simulink model "InductionHeating_bb_4"  (R2026b)
settings: Solver=FixedStepDiscrete  StopTime=0.008
PostLoadFcn:
  | Ts = 1e-6;Ts_fpga=10e-9;   R=3; Capa=300e-9;L=100e-6;Pejo_factor=1;
InitFcn:
  | Ts = 1e-6;Ts_fpga=10e-9;   R=3; Capa=300e-9;L=100e-6;Pejo_factor=1;
undefined symbols (not defined in the file or in its folder): DiscIntNeverNeededParam, ee_sli_rtmsupport, gcbh, isSetWhenUndefinedState, MATESOCwDio
libraries: fl_lib x67, nesl_utility x40, hdlsllib x32, simulink x15, eeGeneralControl x9, ee_lib x3
(part 4 of 7)

== system InductionHeating_bb_4/MATEwDiode/Diode1 ==
  Pejovic L-C-switch component : Subsystem  AncestorBlock=simetranss/FPGA/Pejovic L-C-switch component  mask(Pejovic Element for FPGA simulation){typ=Switch, Lon=LON, L=1, C=1, traprule=off, otherSW='coming soon', Ts=Ts, pcbp=off, showV=on, showI=on}
      mask prompts: typ "Element type"; Lon "Switch equivalent ON inductance (H)"; L "Inductor inductance (H)"; C "Capacitor capacitance (F)"; traprule "Use Trapezoidal rule (LC only)"; otherSW "Linked Compensated switch name"; Ts "Sample Time (s)"; pcbp "Precharge bypass (inverter only)"; showV "Show voltage port"; showI "Show current port"
      mask help:
      | Pejovic L-C-Switch element  in SimScape
      |
      | Implements either  an inductor, a capacitor or a switch using the Pejovic constant admittance method.
      |
      | For the Switch option, the user only has to select the equivalent ON-state inductance of the model, the corresponding Capacitance is computed internally. In the Pejovic model, Ts/Lon=Coff/Ts (Backward Euler) resulting in a constant admittance for the DAE solver.
      |
      |
      | Input signals;
      |
      | gate: the switch gate value (1 for ON , 0 for OFF) (with Switch option)
      mask init:
      | block=gcb;
      | Xcomp=0;
      | s1=0;s2=0;s3=0;s4=0;r1=0;r2=0;l1=0;l2=0;
      | c1=0;c2=0;c3=0;c4=0;x1=0;x2=0;x3=0;x4=0;
      | 
      | MaskEnables =get_param (block ,'MaskEnables' ); 
      | if isequal(get_param(block,"traprule"),'on')
      |     Trapfactor=2;
      | else
      |     Trapfactor=1;
      | end
      | 
      | if isequal(get_param(block,"showV"),'on')
      |         replace_block (block ,'Followlinks' ,'on' ,'Name' ,'v' ,'BlockType' ,'Terminator' ,'Outport' ,'noprompt' ); 
      | else
      |         replace_block (block ,'Followlinks' ,'on' ,'Name' ,'v' ,'BlockType' ,'Outport' ,'Terminator' ,'noprompt' ); 
      | end
      | if isequal(get_param(block,"showI"),'on')
      |         replace_block (block ,'Followlinks' ,'on' ,'Name' ,'i' ,'BlockType' ,'Terminator' ,'Outport' ,'noprompt' ); 
      | else
      |         replace_block (block ,'Followlinks' ,'on' ,'Name' ,'i' ,'BlockType' ,'Outport' ,'Terminator' ,'noprompt' ); 
      | end
      | 
      | 
      | 
      | 
      | 
      | set_param (block ,'MaskEnables' ,MaskEnables ); 
      | qq='Pejo';
      | 
      | typp=get_param(block,'typ');
      | bp=get_param(block,'pcbp');
      | if isequal(typp,'Switch')
      |     replace_block (block ,'Followlinks' ,'on' ,'Name' ,'gate' ,'BlockType' ,'Constant' ,'Inport' ,'noprompt' ); 
      |     replace_block (block ,'Followlinks' ,'on' ,'Name' ,'init_in' ,'BlockType' ,'Inport' ,'Constant' ,'noprompt'  );
      |     replace_block (block ,'Followlinks' ,'on' ,'Name' ,'init_out' ,'BlockType' ,'Outport' ,'Terminator' ,'noprompt'  );
      |     Rsw=Lon/Ts;
      |     txt='Switch';
      |     [s1,s2,s3,s4,r1,r2,l1,l2,c1,c2,c3,c4] = MATEdrawRLC('Series RLC Branch',0,1,0,'Open circuit');
      |     c2=[0 -20];
      |     c1=[30 120];
      |     qq='Pejo Sw';
      | MaskEnables {2 }='on' ; 
      | MaskEnables {3 }='off' ; 
      | MaskEnables {4 }='off' ; 
      | MaskEnables {5 }='off' ; 
      | MaskEnables {6 }='off' ; 
      | MaskEnables {8 }='off' ;
      | %force Backward Euler
      | set_param(block,'traprule','off');
      |  
      | elseif isequal(typp,'Inductor')
      |     replace_block (block ,'Followlinks' ,'on' ,'Name' ,'gate' ,'BlockType' ,'Inport' ,'Constant' ,'noprompt' ); 
      |     set_param([block '/gate'],'Value','1');
      |     replace_block (block ,'Followlinks' ,'on' ,'Name' ,'init_in' ,'BlockType' ,'Inport' ,'Constant' ,'noprompt'  ); 
      |     replace_block (block ,'Followlinks' ,'on' ,'Name' ,'init_out' ,'BlockType' ,'Outport' ,'Terminator' ,'noprompt'  );
      |     Rsw=L/Ts*Trapfactor;
      |     txt='L';
      |     qq='Pejo L';
      | MaskEnables {2 }='off' ; 
      | MaskEnables {3 }='on' ; 
      | MaskEnables {4 }='off' ; 
      | MaskEnables {5 }='on' ; 
      | MaskEnables {6 }='off' ; 
      | MaskEnables {8 }='off' ;
      |     x1=0;x2=0;x3=0;x4=0;
      |     [s1,s2,s3,s4,r1,r2,l1,l2,c1,c2,c3,c4] = MATEdrawRLC('Series RLC Branch',0,1,0,'L');
      |     
      | elseif isequal(typp,'Capacitor')
      |     replace_block (block ,'Followlinks' ,'on' ,'Name' ,'gate' ,'BlockType' ,'Inport' ,'Constant' ,'noprompt' ); 
      |     set_param([block '/gate'],'Value','0');
      |     replace_block (block ,'Followlinks' ,'on' ,'Name' ,'init_in' ,'BlockType' ,'Inport' ,'Constant' ,'noprompt'  );
      |     replace_block (block ,'Followlinks' ,'on' ,'Name' ,'init_out' ,'BlockType' ,'Outport' ,'Terminator' ,'noprompt'  );
      |     Rsw=Ts/C/Trapfactor;
      |     txt='C';
      |     qq='Pejo C';
      | MaskEnables {2 }='off' ; 
      | MaskEnables {3 }='off' ; 
      | MaskEnables {4 }='on' ; 
      | MaskEnables {5 }='on' ; 
      | MaskEnables {6 }='off' ; 
      | MaskEnables {8 }='off' ;
      |         x1=0;x2=0;x3=0;x4=0;
      |     [s1,s2,s3,s4,r1,r2,l1,l2,c1,c2,c3,c4] = MATEdrawRLC('Series RLC Branch',0,0,1,'C');
      | elseif isequal(typp,'2-level inverter switch')
      |     replace_block (block ,'Followlinks' ,'on' ,'Name' ,'gate' ,'BlockType' ,'Constant' ,'Inport' ,'noprompt' ); 
      |     replace_block (block ,'Followlinks' ,'on' ,'Name' ,'init_in' ,'BlockType' ,'Constant' ,'Inport','noprompt'  );
      |     replace_block (block ,'Followlinks' ,'on' ,'Name' ,'init_out' ,'BlockType' ,'Terminator' ,'Outport' ,'noprompt'  );
      |     Rsw=Lon/Ts;
      |     txt='Inverter half';
      |     Xcomp=1;
      |     qq='Pejo Inverter Half';
      |     %force Backward Euler
      | set_param(block,'traprule','off');
      | MaskEnables {2 }='on' ; 
      | MaskEnables {3 }='off' ; 
      | MaskEnables {4 }='off' ; 
      | MaskEnables {5 }='off' ; 
      | MaskEnables {6 }='off' ; 
      | MaskEnables {8 }='on' ;
      |         [s1,s2,s3,s4,r1,r2,l1,l2,c1,c2,c3,c4] = MATEdrawRLC('Series RLC Branch',0,1,0,'Open circuit');
      |     c2=[0 -20];
      |     c1=[30 120];
      | 
      | else
      | end
      | 
      | if isequal(typp,'2-level inverter switch')  && isequal(bp,'on')
      |         replace_block (block ,'Followlinks' ,'on' ,'Name' ,'Bypass' ,'BlockType' ,'Ground' ,'Inport' ,'noprompt' ); 
      | else
      |         replace_block (block ,'Followlinks' ,'on' ,'Name' ,'Bypass' ,'BlockType' ,'Inport' ,'Ground' ,'noprompt' ); 
      | end
      | 
      | MaskEnables {7 }='on' ; 
      | set_param (block ,'MaskEnables' ,MaskEnables ); 
      | 
      | 
      | if Ts>2e-6
      |     %warndlg(['Sample Time of ' num2str(Ts) ' s. may be somehow large for the Pejovic switch to be accurate. Sample time below 2 us are recommended.'])
      | end
      mask TypeOptions typ: Switch | Inductor | Capacitor | 2-level inverter switch
      mask Display:
      | plot(s1,s2,s3,s4,r1,r2,l1,l2,c1,c2,c3,c4,x1,x2,x3,x4);
      | color('blue')
      | port_label('LConn',1,'+')
      | disp([qq  10 10])
  Relational Operator : RelationalOperator  Operator=>  OutDataTypeStr=boolean  RndMeth=Simplest  InputSameDT=off
  Relational Operator1 : RelationalOperator  Operator=>  OutDataTypeStr=boolean  RndMeth=Simplest  InputSameDT=off
  Resistor1 : fl_lib/Electrical/Electrical Elements/Resistor  R=RON Ohm  i_specify=off  i_priority=None  i=0 A  i_nominal_specify=off  i_nominal_value=1  i_nominal_unit=A  v_specify=off  v_priority=None  v=0 V  v_nominal_specify=off  v_nominal_value=1  v_nominal_unit=V
  Set-Reset Flip-Flop : eeGeneralControl/Set-Reset Flip-Flop  LabelModeActiveChoice=Discrete  UndefState=Set  Q0=0  Ts=Ts
  Terminator : Terminator
  Unit Delay : UnitDelay  SampleTime=Ts
  Vf : Constant  Value=0  SampleTime=Ts
  Vf2 : Constant  Value=VF  SampleTime=Ts
  currrent OFF : Constant  Value=0  SampleTime=Ts
  +V : PMIOPort  Side=Left
  -V : PMIOPort  Port=2  Side=Right
  wires:
  Vf2/1 -> Pejovic L-C-switch component/2(Vf)
  Relational Operator/1 -> Set-Reset Flip-Flop/1
  Set-Reset Flip-Flop/1 -> Unit Delay/1
  Unit Delay/1 -> Pejovic L-C-switch component/1(gate)
  Relational Operator1/1 -> Set-Reset Flip-Flop/2
  currrent OFF/1 -> Relational Operator1/2
  Set-Reset Flip-Flop/2 -> Terminator/1
  Vf/1 -> Relational Operator/2
  Pejovic L-C-switch component/2(i) -> Relational Operator1/1
  Pejovic L-C-switch component/1(v) -> Relational Operator/1
  connections:
  Resistor1/RConn1 -- +V/RConn1
  Pejovic L-C-switch component/RConn1 -- -V/RConn1
  Resistor1/LConn1 -- Pejovic L-C-switch component/LConn1

== system InductionHeating_bb_4/MATEwDiode/Diode2 ==
  Pejovic L-C-switch component : Subsystem  AncestorBlock=simetranss/FPGA/Pejovic L-C-switch component  mask(Pejovic Element for FPGA simulation){typ=Switch, Lon=LON, L=1, C=1, traprule=off, otherSW='coming soon', Ts=Ts, pcbp=off, showV=on, showI=on}
      mask prompts: typ "Element type"; Lon "Switch equivalent ON inductance (H)"; L "Inductor inductance (H)"; C "Capacitor capacitance (F)"; traprule "Use Trapezoidal rule (LC only)"; otherSW "Linked Compensated switch name"; Ts "Sample Time (s)"; pcbp "Precharge bypass (inverter only)"; showV "Show voltage port"; showI "Show current port"
      mask help:
      | Pejovic L-C-Switch element  in SimScape
      |
      | Implements either  an inductor, a capacitor or a switch using the Pejovic constant admittance method.
      |
      | For the Switch option, the user only has to select the equivalent ON-state inductance of the model, the corresponding Capacitance is computed internally. In the Pejovic model, Ts/Lon=Coff/Ts (Backward Euler) resulting in a constant admittance for the DAE solver.
      |
      |
      | Input signals;
      |
      | gate: the switch gate value (1 for ON , 0 for OFF) (with Switch option)
      mask init: same as InductionHeating_bb_4/MATEwDiode/Diode1/Pejovic L-C-switch component
      mask TypeOptions typ: Switch | Inductor | Capacitor | 2-level inverter switch
      mask Display:
      | plot(s1,s2,s3,s4,r1,r2,l1,l2,c1,c2,c3,c4,x1,x2,x3,x4);
      | color('blue')
      | port_label('LConn',1,'+')
      | disp([qq  10 10])
  Relational Operator : RelationalOperator  Operator=>  OutDataTypeStr=boolean  RndMeth=Simplest  InputSameDT=off
  Relational Operator1 : RelationalOperator  Operator=>  OutDataTypeStr=boolean  RndMeth=Simplest  InputSameDT=off
  Resistor1 : fl_lib/Electrical/Electrical Elements/Resistor  R=RON Ohm  i_specify=off  i_priority=None  i=0 A  i_nominal_specify=off  i_nominal_value=1  i_nominal_unit=A  v_specify=off  v_priority=None  v=0 V  v_nominal_specify=off  v_nominal_value=1  v_nominal_unit=V
  Set-Reset Flip-Flop : eeGeneralControl/Set-Reset Flip-Flop  LabelModeActiveChoice=Discrete  UndefState=Set  Q0=0  Ts=Ts
  Terminator : Terminator
  Unit Delay : UnitDelay  SampleTime=Ts
  Vf : Constant  Value=0  SampleTime=Ts
  Vf2 : Constant  Value=VF  SampleTime=Ts
  currrent OFF : Constant  Value=0  SampleTime=Ts
  +V : PMIOPort  Side=Left
  -V : PMIOPort  Port=2  Side=Right
  wires:
  Pejovic L-C-switch component/1(v) -> Relational Operator/1
  Pejovic L-C-switch component/2(i) -> Relational Operator1/1
  Vf/1 -> Relational Operator/2
  Set-Reset Flip-Flop/2 -> Terminator/1
  currrent OFF/1 -> Relational Operator1/2
  Relational Operator1/1 -> Set-Reset Flip-Flop/2
  Unit Delay/1 -> Pejovic L-C-switch component/1(gate)
  Set-Reset Flip-Flop/1 -> Unit Delay/1
  Relational Operator/1 -> Set-Reset Flip-Flop/1
  Vf2/1 -> Pejovic L-C-switch component/2(Vf)
  connections:
  Resistor1/LConn1 -- Pejovic L-C-switch component/LConn1
  Pejovic L-C-switch component/RConn1 -- -V/RConn1
  Resistor1/RConn1 -- +V/RConn1

== system InductionHeating_bb_4/MATEwDiode/Diode3 ==
  Pejovic L-C-switch component : Subsystem  AncestorBlock=simetranss/FPGA/Pejovic L-C-switch component  mask(Pejovic Element for FPGA simulation){typ=Switch, Lon=LON, L=1, C=1, traprule=off, otherSW='coming soon', Ts=Ts, pcbp=off, showV=on, showI=on}
      mask prompts: typ "Element type"; Lon "Switch equivalent ON inductance (H)"; L "Inductor inductance (H)"; C "Capacitor capacitance (F)"; traprule "Use Trapezoidal rule (LC only)"; otherSW "Linked Compensated switch name"; Ts "Sample Time (s)"; pcbp "Precharge bypass (inverter only)"; showV "Show voltage port"; showI "Show current port"
      mask help:
      | Pejovic L-C-Switch element  in SimScape
      |
      | Implements either  an inductor, a capacitor or a switch using the Pejovic constant admittance method.
      |
      | For the Switch option, the user only has to select the equivalent ON-state inductance of the model, the corresponding Capacitance is computed internally. In the Pejovic model, Ts/Lon=Coff/Ts (Backward Euler) resulting in a constant admittance for the DAE solver.
      |
      |
      | Input signals;
      |
      | gate: the switch gate value (1 for ON , 0 for OFF) (with Switch option)
      mask init: same as InductionHeating_bb_4/MATEwDiode/Diode1/Pejovic L-C-switch component
      mask TypeOptions typ: Switch | Inductor | Capacitor | 2-level inverter switch
      mask Display:
      | plot(s1,s2,s3,s4,r1,r2,l1,l2,c1,c2,c3,c4,x1,x2,x3,x4);
      | color('blue')
      | port_label('LConn',1,'+')
      | disp([qq  10 10])
  Relational Operator : RelationalOperator  Operator=>  OutDataTypeStr=boolean  RndMeth=Simplest  InputSameDT=off
  Relational Operator1 : RelationalOperator  Operator=>  OutDataTypeStr=boolean  RndMeth=Simplest  InputSameDT=off
  Resistor1 : fl_lib/Electrical/Electrical Elements/Resistor  R=RON Ohm  i_specify=off  i_priority=None  i=0 A  i_nominal_specify=off  i_nominal_value=1  i_nominal_unit=A  v_specify=off  v_priority=None  v=0 V  v_nominal_specify=off  v_nominal_value=1  v_nominal_unit=V
  Set-Reset Flip-Flop : eeGeneralControl/Set-Reset Flip-Flop  LabelModeActiveChoice=Discrete  UndefState=Set  Q0=0  Ts=Ts
  Terminator : Terminator
  Unit Delay : UnitDelay  SampleTime=Ts
  Vf : Constant  Value=0  SampleTime=Ts
  Vf2 : Constant  Value=VF  SampleTime=Ts
  currrent OFF : Constant  Value=0  SampleTime=Ts
  +V : PMIOPort  Side=Left
  -V : PMIOPort  Port=2  Side=Right
  wires:
  Pejovic L-C-switch component/1(v) -> Relational Operator/1
  Pejovic L-C-switch component/2(i) -> Relational Operator1/1
  Vf/1 -> Relational Operator/2
  Set-Reset Flip-Flop/2 -> Terminator/1
  currrent OFF/1 -> Relational Operator1/2
  Relational Operator1/1 -> Set-Reset Flip-Flop/2
  Unit Delay/1 -> Pejovic L-C-switch component/1(gate)
  Set-Reset Flip-Flop/1 -> Unit Delay/1
  Relational Operator/1 -> Set-Reset Flip-Flop/1
  Vf2/1 -> Pejovic L-C-switch component/2(Vf)
  connections:
  Resistor1/LConn1 -- Pejovic L-C-switch component/LConn1
  Pejovic L-C-switch component/RConn1 -- -V/RConn1
  Resistor1/RConn1 -- +V/RConn1

== system InductionHeating_bb_4/MATEwDiode/Diode4 ==
  Pejovic L-C-switch component : Subsystem  AncestorBlock=simetranss/FPGA/Pejovic L-C-switch component  mask(Pejovic Element for FPGA simulation){typ=Switch, Lon=LON, L=1, C=1, traprule=off, otherSW='coming soon', Ts=Ts, pcbp=off, showV=on, showI=on}
      mask prompts: typ "Element type"; Lon "Switch equivalent ON inductance (H)"; L "Inductor inductance (H)"; C "Capacitor capacitance (F)"; traprule "Use Trapezoidal rule (LC only)"; otherSW "Linked Compensated switch name"; Ts "Sample Time (s)"; pcbp "Precharge bypass (inverter only)"; showV "Show voltage port"; showI "Show current port"
      mask help:
      | Pejovic L-C-Switch element  in SimScape
      |
      | Implements either  an inductor, a capacitor or a switch using the Pejovic constant admittance method.
      |
      | For the Switch option, the user only has to select the equivalent ON-state inductance of the model, the corresponding Capacitance is computed internally. In the Pejovic model, Ts/Lon=Coff/Ts (Backward Euler) resulting in a constant admittance for the DAE solver.
      |
      |
      | Input signals;
      |
      | gate: the switch gate value (1 for ON , 0 for OFF) (with Switch option)
      mask init: same as InductionHeating_bb_4/MATEwDiode/Diode1/Pejovic L-C-switch component
      mask TypeOptions typ: Switch | Inductor | Capacitor | 2-level inverter switch
      mask Display:
      | plot(s1,s2,s3,s4,r1,r2,l1,l2,c1,c2,c3,c4,x1,x2,x3,x4);
      | color('blue')
      | port_label('LConn',1,'+')
      | disp([qq  10 10])
  Relational Operator : RelationalOperator  Operator=>  OutDataTypeStr=boolean  RndMeth=Simplest  InputSameDT=off
  Relational Operator1 : RelationalOperator  Operator=>  OutDataTypeStr=boolean  RndMeth=Simplest  InputSameDT=off
  Resistor1 : fl_lib/Electrical/Electrical Elements/Resistor  R=RON Ohm  i_specify=off  i_priority=None  i=0 A  i_nominal_specify=off  i_nominal_value=1  i_nominal_unit=A  v_specify=off  v_priority=None  v=0 V  v_nominal_specify=off  v_nominal_value=1  v_nominal_unit=V
  Set-Reset Flip-Flop : eeGeneralControl/Set-Reset Flip-Flop  LabelModeActiveChoice=Discrete  UndefState=Set  Q0=0  Ts=Ts
  Terminator : Terminator
  Unit Delay : UnitDelay  SampleTime=Ts
  Vf : Constant  Value=0  SampleTime=Ts
  Vf2 : Constant  Value=VF  SampleTime=Ts
  currrent OFF : Constant  Value=0  SampleTime=Ts
  +V : PMIOPort  Side=Left
  -V : PMIOPort  Port=2  Side=Right
  wires:
  Vf2/1 -> Pejovic L-C-switch component/2(Vf)
  Relational Operator/1 -> Set-Reset Flip-Flop/1
  Set-Reset Flip-Flop/1 -> Unit Delay/1
  Unit Delay/1 -> Pejovic L-C-switch component/1(gate)
  Relational Operator1/1 -> Set-Reset Flip-Flop/2
  currrent OFF/1 -> Relational Operator1/2
  Set-Reset Flip-Flop/2 -> Terminator/1
  Vf/1 -> Relational Operator/2
  Pejovic L-C-switch component/2(i) -> Relational Operator1/1
  Pejovic L-C-switch component/1(v) -> Relational Operator/1
  connections:
  Resistor1/RConn1 -- +V/RConn1
  Pejovic L-C-switch component/RConn1 -- -V/RConn1
  Resistor1/LConn1 -- Pejovic L-C-switch component/LConn1

== system InductionHeating_bb_4/MATEwDiode/MATE 2-level inverter ==
  g : Inport
  CCS_Idc : fl_lib/Electrical/Electrical Sources/Controlled Current Source
  CVS : fl_lib/Electrical/Electrical Sources/Controlled Voltage Source
  Constant : Constant  Value=[Gpp Ts/Gip min_charge Vf]  SampleTime=Ts
  Isensor : fl_lib/Electrical/Electrical Sensors/Current Sensor
  PS-Simulink Converter : nesl_utility/PS-Simulink Converter  PhysicalDomain=network_engine_domain  SubClassName=ps_output  LeftPortType=input  RightPortType=output  PseudoPeriodic=off  Frequencies=[]  VectorFormat=inherit  Unit=inherit  AffineConversion=off
  PS-Simulink Converter1 : nesl_utility/PS-Simulink Converter  PhysicalDomain=network_engine_domain  SubClassName=ps_output  LeftPortType=input  RightPortType=output  PseudoPeriodic=off  Frequencies=[]  VectorFormat=inherit  Unit=inherit  AffineConversion=off
  R : fl_lib/Electrical/Electrical Elements/Resistor  R=Ron Ohm  i_specify=off  i_priority=None  i=0 A  i_nominal_specify=off  i_nominal_value=1  i_nominal_unit=A  v_specify=off  v_priority=None  v=0 V  v_nominal_specify=off  v_nominal_value=1  v_nominal_unit=V
  SW : Subsystem
  Selector : Selector  InputPortWidth=2  IndexOptions=Index vector (dialog)  Indices=[1 ]  OutputSizes=1  RuntimeRangeChecks=off
  Selector1 : Selector  InputPortWidth=2  IndexOptions=Index vector (dialog)  Indices=[2 ]  OutputSizes=1  RuntimeRangeChecks=off
  Simulink-PS Converter : nesl_utility/Simulink-PS Converter  PhysicalDomain=network_engine_domain  SubClassName=ps_input  LeftPortType=input  RightPortType=output  PseudoPeriodic=off  Frequencies=[]  NoiseDistribution=none  NoiseParameters=[]  Unit=1  AffineConversion=off  FilteringAndDerivatives=provide  SimscapeFilterOrder=1  InputFilterTimeConstant=0.001  UdotUserProvided=0
  Simulink-PS Converter1 : nesl_utility/Simulink-PS Converter  PhysicalDomain=network_engine_domain  SubClassName=ps_input  LeftPortType=input  RightPortType=output  PseudoPeriodic=off  Frequencies=[]  NoiseDistribution=none  NoiseParameters=[]  Unit=1  AffineConversion=off  FilteringAndDerivatives=provide  SimscapeFilterOrder=1  InputFilterTimeConstant=0.001  UdotUserProvided=0
  Unit Delay2 : UnitDelay  SampleTime=Ts
  Unit Delay3 : UnitDelay  SampleTime=Ts
  Vsensor : fl_lib/Electrical/Electrical Sensors/Voltage Sensor
  V+ : PMIOPort  Side=Left
  V- : PMIOPort  Port=2  Side=Left
  A : PMIOPort  Port=3  Side=Right
  wires:
  SW/2(Vac) -> Simulink-PS Converter1/1
  Constant/1 -> SW/5(params)
  Unit Delay3/1 -> SW/3(Vdc)
  Unit Delay2/1 -> SW/4(Iac)
  SW/1(Idc) -> Simulink-PS Converter/1
  g/1 -> Selector/1, Selector1/1
  PS-Simulink Converter1/1 -> Unit Delay3/1
  PS-Simulink Converter/1 -> Unit Delay2/1
  Selector/1 -> SW/1(gu)
  Selector1/1 -> SW/2(gl)
  connections:
  Isensor/RConn2 -- CVS/LConn1
  R/LConn1 -- Isensor/LConn1
  Simulink-PS Converter/RConn1 -- CCS_Idc/RConn1
  PS-Simulink Converter/LConn1 -- Isensor/RConn1
  Simulink-PS Converter1/RConn1 -- CVS/RConn1
  CCS_Idc/LConn1 -- Vsensor/RConn2 -- V-/RConn1 -- CVS/RConn2
  CCS_Idc/RConn2 -- Vsensor/LConn1 -- V+/RConn1
  PS-Simulink Converter1/LConn1 -- Vsensor/RConn1
  A/RConn1 -- R/RConn1

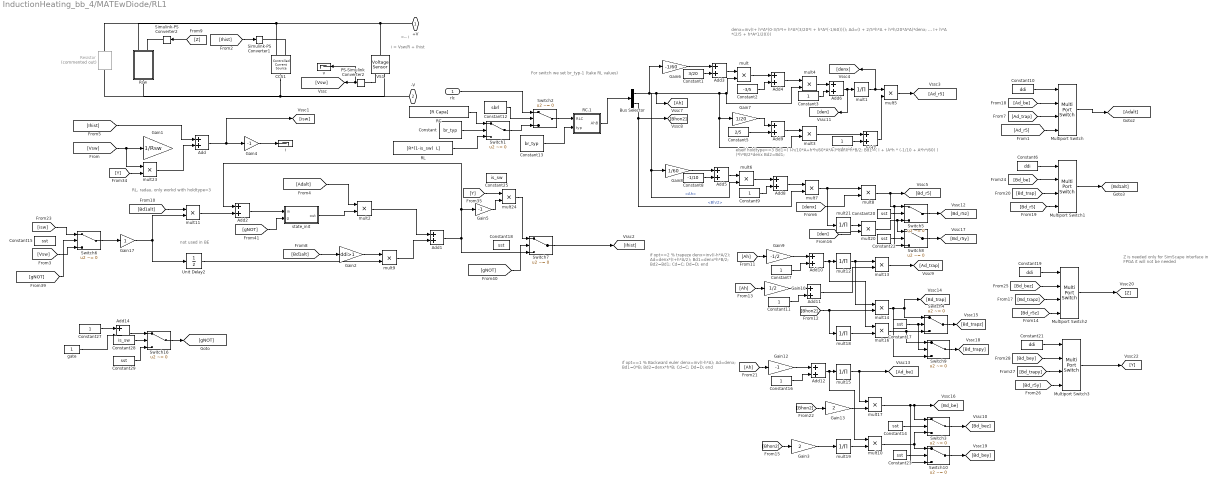
== system InductionHeating_bb_4/MATEwDiode/RL1 ==
  note: For switch we set br_typ-1 (take RL values)
  note: if opt==1 % Backward euler
      | denx=inv(I-h*A);
      | Ad=denx;
      | Bd1=0*B;
      | Bd2=denx*h*B;
      | Cd=C;
      | Dd=D;
      | end
  note: if opt==2 % trapeze
      | denx=inv(I-h*A/2);
      | Ad=denx*(I+h*A/2);
      | Bd1=denx*h*B/2;
      | Bd2=Bd1;
      | Cd=C;
      | Dd=D;
      | end
  note: RL, radau, only workd with holdtype=3
  note: elseif holdtype==3
      | Bd1=( I-h/10*A+h*h/60*A*A )*denx*h*B/2;
      | Bd1=( I + (A*h * (-1/10 + A*h*/60) ) )*h*B/2*denx
      | Bd2=Bd1;
  note: denx=inv(I+ h*A*(0-3/5*I+ h*A*(3/20*I + h*A*(-1/60))));
      | Ad=(I + 2/5*h*A + h*h/20*A*A)*denx;
      | ... I+ h*A *(2/5 + h*A*1/20)))
  note: <-- i
  note: i = Vsw/R + Ihist
  note: Z is needed only for SimScape interface
      | in FPGA it will not be needed
  note: not used in BE
  rlc : Inport
  Add : Sum
  Add{1..12} (12 alike) : Sum  Inputs=2
  Add14 : Sum  Inputs=+-
  Bus Selector : BusSelector  OutputSignals=Ah,Bh/2
  CCS1 : fl_lib/Electrical/Electrical Sources/Controlled Current Source
  Constant : Constant  Value=br_typ
  Constant1 : Constant  Value=3/20  SampleTime=Ts
  Constant{6,10,19,21} (4 alike) : Constant  Value=ddi  SampleTime=Ts
  Constant{3..4,7,9,11,16,27} (7 alike) : Constant  SampleTime=Ts
  Constant12 : Constant  Value=sbrl
  Constant13 : Constant  Value=br_typ
  Constant{14..15,17..18,20,22..23,29} (8 alike) : Constant  Value=sst  SampleTime=Ts
  Constant2 : Constant  Value=-3/5  SampleTime=Ts
  Constant25 : Constant  Value=is_sw  SampleTime=Ts
  Constant28 : Constant  Value=is_sw  SampleTime=Ts
  Constant5 : Constant  Value=2/5  SampleTime=Ts
  Constant8 : Constant  Value=-1/10  SampleTime=Ts
  Gain1 : Gain  Gain=1/Rsw
  Gain10 : Gain  Gain=1/2
  Gain12 : Gain  Gain=-1
  Gain13 : Gain  Gain=2
  Gain17 : Gain
  Gain2 : Gain  Gain=ddi>1
  Gain3 : Gain  Gain=2
  Gain4 : Gain  Gain=-1
  Gain5 : Gain  Gain=-1
  Gain6 : Gain  Gain=-1/60
  Gain7 : Gain  Gain=1/20
  Gain8 : Gain  Gain=1/60
  Gain9 : Gain  Gain=-1/2
  Multiport Switch{,1..3} (4 alike) : MultiPortSwitch  SaturateOnIntegerOverflow=off  InputSameDT=off
  PS-Simulink Converter2 : nesl_utility/PS-Simulink Converter  PhysicalDomain=network_engine_domain  SubClassName=ps_output  LeftPortType=input  RightPortType=output  PseudoPeriodic=off  Frequencies=[]  VectorFormat=inherit  Unit=inherit  AffineConversion=off
  RC : Constant  Value=[R Capa]  SampleTime=Ts
  RC.1 : Subsystem
  RL : Constant  Value="[R*(1-is_sw)  L]"  SampleTime=Ts
  Resistor : fl_lib/Electrical/Electrical Elements/Resistor  Commented=on  R=Rsw Ohm  i_specify=off  i_priority=None  i=0 A  i_nominal_specify=off  i_nominal_value=1  i_nominal_unit=A  v_specify=off  v_priority=None  v=0 V  v_nominal_specify=off  v_nominal_value=1  v_nominal_unit=V
  Rsw : Subsystem  mask(Simscape MATE variable resistance default value mask){defaultR=Rsw}
      mask prompts: defaultR "Default Resistance"
  Simulink-PS Converter1 : nesl_utility/Simulink-PS Converter  PhysicalDomain=network_engine_domain  SubClassName=ps_input  LeftPortType=input  RightPortType=output  PseudoPeriodic=off  Frequencies=[]  NoiseDistribution=none  NoiseParameters=[]  Unit=1  AffineConversion=off  FilteringAndDerivatives=provide  SimscapeFilterOrder=1  InputFilterTimeConstant=0.001  UdotUserProvided=0
  Simulink-PS Converter2 : nesl_utility/Simulink-PS Converter  PhysicalDomain=network_engine_domain  SubClassName=ps_input  LeftPortType=input  RightPortType=output  PseudoPeriodic=off  Frequencies=[]  NoiseDistribution=none  NoiseParameters=[]  Unit=1  AffineConversion=off  FilteringAndDerivatives=provide  SimscapeFilterOrder=1  InputFilterTimeConstant=0.001  UdotUserProvided=0
  Switch{1..10} (10 alike) : Switch  Criteria=u2 ~= 0  SaturateOnIntegerOverflow=off  InputSameDT=off
  Switch16 : Switch  Criteria=u2 ~= 0  Threshold=0.5  SaturateOnIntegerOverflow=off  InputSameDT=off
  Unit Delay2 : UnitDelay  SampleTime=-1
  VS1 : fl_lib/Electrical/Electrical Sensors/Voltage Sensor
  gate : Constant
  i : Terminator
  mult{,2..11,13..14,16..17,20,23..24} (18 alike) : Product
  mult{1,12,15,18..19,21} (6 alike) : Product  Inputs=/
  state_init : Subsystem
  v : Terminator
  +V : PMIOPort  Side=Left
  -V : PMIOPort  Port=2  Side=Right
  wires:
  Constant29/1 -> Switch16/3
  Constant28/1 -> Switch16/2
  Switch16/1 -> [gNOT]
  Add14/1 -> Switch16/1
  [gNOT] -> state_init/2(g)
  state_init/1(out) -> mult2/2
  [gNOT] -> Switch7/2
  [gNOT] -> Switch6/2
  Constant27/1 -> Add14/1
  Gain17/1 -> Unit Delay2/1, mult11/2
  Gain5/1 -> mult24/2
  [Y] -> mult24/1
  mult24/1 -> Switch7/1
  mult23/1 -> Add/2
  [Y] -> mult23/2
  Multiport Switch3/1 -> [Y]
  Constant23/1 -> Switch10/2
  Switch10/1 -> [Bd_bey]
  mult14/1 -> Switch4/1, [Bd_trap], Switch9/3
  mult16/1 -> Switch4/3, Switch9/1
  Constant17/1 -> Switch4/2, Switch9/2
  Switch9/1 -> [Bd_trapy]
  Constant22/1 -> Switch8/2
  Switch8/1 -> [Bd_r5y]
  [Bd_r5y] -> Multiport Switch3/4
  [Bd_trapy] -> Multiport Switch3/3
  [Bd_bey] -> Multiport Switch3/2
  Constant21/1 -> Multiport Switch3/1
  Switch4/1 -> [Bd_trapz]
  mult8/1 -> Switch5/1, Switch8/3, [Bd_r5]
  Constant19/1 -> Multiport Switch2/1
  Multiport Switch2/1 -> [Z]
  [Bd_bez] -> Multiport Switch2/2
  [Bd_trapz] -> Multiport Switch2/3
  [Bd_r5z] -> Multiport Switch2/4
  mult2/1 -> Add1/1
  [isw] -> Switch6/1
  [Vsw] -> Switch6/3
  Switch6/1 -> Gain17/1
  Add/1 -> Gain4/1, [isw]
  [Ihist] -> Simulink-PS Converter1/1
  [Vsw] -> Gain1/1, mult23/1
  PS-Simulink Converter2/1 -> v/1, [Vsw]
  [Ihist] -> Add/1
  Gain4/1 -> i/1
  Add2/1 -> state_init/1(in)
  Add1/1 -> Add2/1, Gain5/1, Switch7/3
  Unit Delay2/1 -> mult9/2
  Gain6/1 -> Add3/1
  Constant1/1 -> Add3/2
  mult/1 -> Add4/1
  Add3/1 -> mult/1
  Constant2/1 -> Add4/2
  Add4/1 -> mult4/1
  mult4/1 -> Add6/1
  Constant3/1 -> Add6/2
  Add6/1 -> [den], mult1/1
  Constant4/1 -> Add7/2
  Constant5/1 -> Add9/2
  Add9/1 -> mult3/1
  Gain7/1 -> Add9/1
  mult3/1 -> Add7/1
  Add7/1 -> mult5/2
  [Adalt] -> mult2/1
  mult1/1 -> [denx], mult5/1
  mult5/1 -> [Ad_r5]
  Constant9/1 -> Add8/2
  Add5/1 -> mult6/1
  mult6/1 -> Add8/1
  Constant8/1 -> Add5/2
  Gain8/1 -> Add5/1
  Add8/1 -> mult7/1
  mult7/1 -> mult21/1, mult8/1
  [denx] -> mult8/2
  Bus Selector/1 -> Gain6/1, [Ah], mult3/2, Gain7/1, mult4/2, mult/2, Gain8/1, mult6/2  "<Ah>"
  Bus Selector/2 -> mult7/2, [Bhon2]  "<Bh/2>"
  [Z] -> Simulink-PS Converter2/1
  [Ah] -> Gain9/1
  Gain9/1 -> Add10/1
  Constant7/1 -> Add10/2
  Add10/1 -> mult16/1, mult12/1
  Add11/1 -> mult13/2
  Constant11/1 -> Add11/2
  Gain10/1 -> Add11/1
  [Ah] -> Gain10/1
  mult12/1 -> mult14/1, mult13/1
  [Bhon2] -> mult18/1, mult14/2
  mult13/1 -> [Ad_trap]
  mult9/1 -> Add1/2
  [Bd1alt] -> Gain2/1
  [Bd1alt] -> mult11/1
  mult11/1 -> Add2/2
  mult15/1 -> [Ad_be], mult17/1
  [Bhon2] -> Gain13/1
  Add12/1 -> mult10/1, mult15/1
  Constant16/1 -> Add12/2
  Gain12/1 -> Add12/1
  [Ah] -> Gain12/1
  Gain13/1 -> mult17/2
  [Ad_r5] -> Multiport Switch/4
  [Ad_trap] -> Multiport Switch/3
  [Ad_be] -> Multiport Switch/2
  Multiport Switch/1 -> [Adalt]
  [Bd_r5] -> Multiport Switch1/4
  [Bd_trap] -> Multiport Switch1/3
  [Bd_be] -> Multiport Switch1/2
  Multiport Switch1/1 -> [Bd1alt]
  Constant6/1 -> Multiport Switch1/1
  Constant10/1 -> Multiport Switch/1
  Gain2/1 -> mult9/1
  RC/1 -> Switch1/1
  RL/1 -> Switch1/3
  Constant/1 -> Switch1/2
  Switch1/1 -> Switch2/3
  Switch2/1 -> RC.1/1(RLC)
  rlc/1 -> Switch2/1
  Constant12/1 -> Switch2/2
  RC.1/1(AhB) -> Bus Selector/1
  Constant13/1 -> RC.1/2(typ)
  mult18/1 -> mult16/2
  Gain3/1 -> mult19/1
  [Bhon2] -> Gain3/1
  mult19/1 -> mult10/2
  mult10/1 -> Switch3/3, Switch10/1
  mult17/1 -> Switch3/1, [Bd_be], Switch10/3
  Constant14/1 -> Switch3/2
  Switch3/1 -> [Bd_bez]
  [den] -> mult20/2
  mult21/1 -> mult20/1
  Switch5/1 -> [Bd_r5z]
  Constant20/1 -> Switch5/2
  mult20/1 -> Switch5/3, Switch8/1
  gate/1 -> Add14/2
  Switch7/1 -> [Ihist]
  connections:
  CCS1/RConn2 -- +V/RConn1 -- VS1/LConn1 -- Resistor/LConn1 -- Rsw/LConn1
  CCS1/RConn1 -- Simulink-PS Converter1/RConn1
  PS-Simulink Converter2/LConn1 -- VS1/RConn1
  CCS1/LConn1 -- -V/RConn1 -- VS1/RConn2 -- Resistor/RConn1 -- Rsw/RConn1
  Simulink-PS Converter2/RConn1 -- Rsw/LConn2

== system InductionHeating_bb_4/MATEwDiode/Subsystem3 ==
  ILoad : fl_lib/Electrical/Electrical Sensors/Current Sensor
  PS-Simulink Converter : nesl_utility/PS-Simulink Converter  PhysicalDomain=network_engine_domain  SubClassName=ps_output  LeftPortType=input  RightPortType=output  PseudoPeriodic=off  Frequencies=[]  VectorFormat=1-D array  Unit=inherit  AffineConversion=off
  + : PMIOPort  Side=Left
  - : PMIOPort  Port=2  Side=Right
  i : Outport
  wires:
  PS-Simulink Converter/1 -> i/1
  connections:
  +/RConn1 -- ILoad/LConn1
  ILoad/RConn2 -- -/RConn1
  PS-Simulink Converter/LConn1 -- ILoad/RConn1

== system InductionHeating_bb_4/PWM_Generator3/Discrete Triangular-Waveform Generator ==
  steps : Inport
  stepON : Inport  Port=2
  Add : Sum  Inputs=+-  OutDataTypeStr=int32
  Add1 : Sum  Inputs=+-  OutDataTypeStr=int32
  Constat : Constant  Value=0  OutDataTypeStr=int32  SampleTime=Ts
  Constat1 : Constant  OutDataTypeStr=int32  SampleTime=Ts
  Constat2 : Constant  Value=0  OutDataTypeStr=int32  SampleTime=Ts
  Constat3 : Constant  OutDataTypeStr=int32  SampleTime=Ts
  Data Type Conversion1 : DataTypeConversion  OutDataTypeStr=int32  RndMeth=Nearest  SaturateOnIntegerOverflow=off
  Data Type Conversion2 : DataTypeConversion  OutDataTypeStr=int32  RndMeth=Nearest  SaturateOnIntegerOverflow=off
  Logical Operator : Logic  AllPortsSameDT=off  OutDataTypeStr=boolean
  Relational Operator2 : RelationalOperator  OutDataTypeStr=boolean
  Relational Operator3 : RelationalOperator  OutDataTypeStr=boolean
  Relational Operator4 : RelationalOperator  Operator=<=  OutDataTypeStr=boolean
  Shift Arithmetic1 : ArithShift  BitShiftNumber=1  BitShiftDirection=Right
  Sum2 : Sum  InputSameDT=on  SaturateOnIntegerOverflow=on  OutDataTypeStr=Inherit: Same as first input
  Switch : Switch  Criteria=u2 ~= 0
  Switch1 : Switch  Criteria=u2 ~= 0
  Unit Delay Enabled Synchronous : hdlsllib/Discrete/Unit Delay Enabled Synchronous  InitialCondition=0.0  SampleTime=-1
  Unit Delay Enabled Synchronous1 : hdlsllib/Discrete/Unit Delay Enabled Synchronous  InitialCondition=0.0  SampleTime=-1
  Unit Delay1 : UnitDelay  SampleTime=Ts
  pulse : Outport  InitialOutput=0  VectorParamsAs1DForOutWhenUnconnected=off
  wires:
  Constat3/1 -> Add1/2
  Add1/1 -> Add/1, Relational Operator3/2
  Unit Delay Enabled Synchronous1/1 -> Data Type Conversion2/1
  Unit Delay Enabled Synchronous/1 -> Data Type Conversion1/1
  stepON/1 -> Unit Delay Enabled Synchronous1/1
  steps/1 -> Unit Delay Enabled Synchronous/1
  Shift Arithmetic1/1 -> Relational Operator2/2, Add/2
  Switch1/1 -> Sum2/2
  Constat2/1 -> Switch1/1
  Add/1 -> Relational Operator4/2
  Logical Operator/1 -> pulse/1
  Relational Operator4/1 -> Logical Operator/2
  Relational Operator2/1 -> Logical Operator/1
  Constat1/1 -> Switch/3
  Data Type Conversion2/1 -> Shift Arithmetic1/1
  Relational Operator3/1 -> Switch1/2, Unit Delay Enabled Synchronous1/2, Unit Delay Enabled Synchronous/2, Switch/2
  Data Type Conversion1/1 -> Add1/1
  Sum2/1 -> Unit Delay1/1, Relational Operator2/1, Relational Operator4/1
  Unit Delay1/1 -> Switch1/3, Relational Operator3/1
  Switch/1 -> Sum2/1
  Constat/1 -> Switch/1

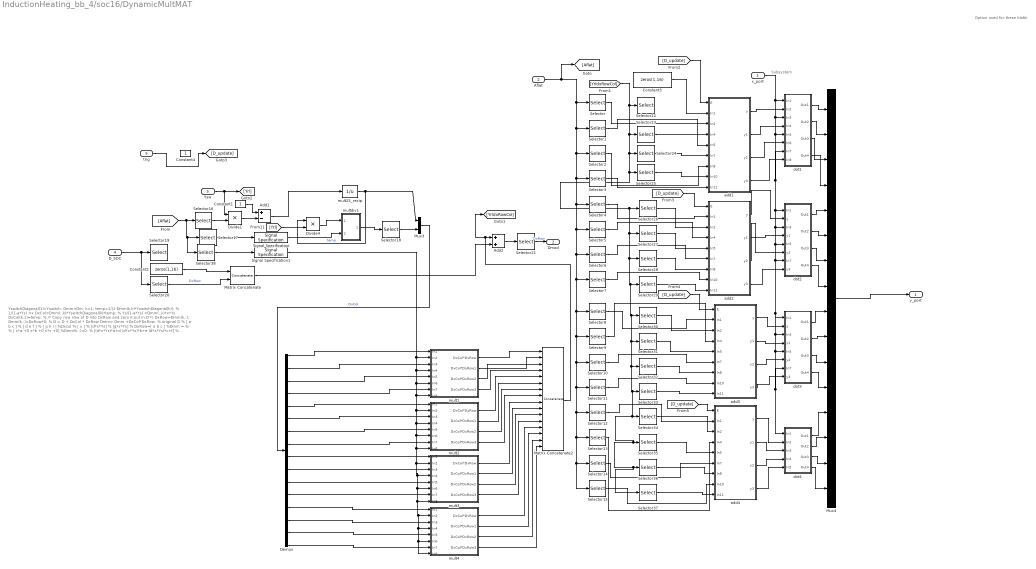
== system InductionHeating_bb_4/soc16/DynamicMultMAT ==
  note: Option used for these blobk
  note: Subsystem
  note: YswitchDiagonal(1)=Yswitch;
      | Dmm=Dm;
      | k=1;
      | temp=1/(1-Dmm(k,k)*YswitchDiagonal(k)); % 1/(1-a*Ys) =x
      | DxCol=Dmm(:,k)*YswitchDiagonal(k)*temp; % Ys/(1-a*Ys) =Dmm(:,k)*x*Ys
      | DxCol(k,1)=temp;
      | % /* Copy row nSw of D into DxRow and zero it out in D */
      | DxRow=Dmm(k,:);
      | Dmm(k,:)=DxRow*0;
      | % D = D + DxCol * DxRow
      | Dmm= Dmm +DxCol*DxRow;
      | % original D
      | % [ a b c ]
      | % [ d e f ]
      | % [ g h i ]
      | %Dxcol
      | % [ x ]
      | % [d*x*Ys]
      | % [g*x*Ys]
      | % DxRow=[ a b c ]
      | %Dmm =
      | % % [ x*a +0 x*b +0 x*c +0] %Dmm(k,:)=0;
      | % [(d*x*Ys)*a+d (d*x*Ys)*b+e (d*x*Ys)*c+f]
      | % [(g*x*Ys)*a+g (g*x*Ys)*b+h (g*x*Ys)*c+i]
  x_port : Inport
  Aflat : Inport  Port=2
  Ysw : Inport  Port=3
  D_SOC : Inport  Port=4
  trig : Inport  Port=5
  Add1 : Sum  Inputs=+-
  Add2 : Sum
  Constant1 : Constant  OutDataTypeStr=single  SampleTime=Ts
  Constant2 : Constant  Value=zeros(1,16)  VectorParams1D=off  OutDataTypeStr=single  SampleTime=Ts
  Constant3 : Constant  Value=zeros(1,16)  OutDataTypeStr=single  SampleTime=Ts
  Constant4 : Constant  OutDataTypeStr=single  SampleTime=Ts
  Demux : Demux  Outputs=16
  Divide1 : Product
  Divide4 : Product
  Matrix Concatenate : Concatenate  Mode=Multidimensional array
  Matrix Concatenate2 : Concatenate  NumInputs=16  Mode=Multidimensional array
  Mux3 : Mux  Inputs=2
  Mux4 : Mux  Inputs=16
  Selector : Selector  InputPortWidth=16*16  IndexOptions=Index vector (dialog)  Indices=[1:16]  OutputSizes=1  RuntimeRangeChecks=off
  Selector1 : Selector  InputPortWidth=16*16  IndexOptions=Index vector (dialog)  Indices=[1:16]+16*1  OutputSizes=1  RuntimeRangeChecks=off
  Selector10 : Selector  InputPortWidth=16*16  IndexOptions=Index vector (dialog)  Indices=[1:16]+16*10  OutputSizes=1  RuntimeRangeChecks=off
  Selector11 : Selector  InputPortWidth=16*16  IndexOptions=Index vector (dialog)  Indices=[1:16]+16*11  OutputSizes=1  RuntimeRangeChecks=off
  Selector12 : Selector  InputPortWidth=16*16  IndexOptions=Index vector (dialog)  Indices=[1:16]+16*12  OutputSizes=1  RuntimeRangeChecks=off
  Selector13 : Selector  InputPortWidth=16*16  IndexOptions=Index vector (dialog)  Indices=[1:16]+16*13  OutputSizes=1  RuntimeRangeChecks=off
  Selector14 : Selector  InputPortWidth=16*16  IndexOptions=Index vector (dialog)  Indices=[1:16]+16*14  OutputSizes=1  RuntimeRangeChecks=off
  Selector15 : Selector  InputPortWidth=16*16  IndexOptions=Index vector (dialog)  Indices=[1:16]+16*15  OutputSizes=1  RuntimeRangeChecks=off
  Selector16 : Selector  InputPortWidth=16*16  IndexOptions=Index vector (dialog)  Indices=[1]  OutputSizes=1  RuntimeRangeChecks=off
  Selector17 : Selector  InputPortWidth=16*16  IndexOptions=Index vector (dialog)  Indices=[1:16:16*16]  OutputSizes=1  RuntimeRangeChecks=off
  Selector18 : Selector  InputPortWidth=16  IndexOptions=Index vector (dialog)  Indices=[2:16]  OutputSizes=1  RuntimeRangeChecks=off
  Selector19 : Selector  NumberOfDimensions=2  InputPortWidth=3  IndexOptions=Index vector (dialog),Index vector (dialog)  Indices=1,[1:16]  OutputSizes=1,1  RuntimeRangeChecks=off
  Selector2 : Selector  InputPortWidth=16*16  IndexOptions=Index vector (dialog)  Indices=[1:16]+16*2  OutputSizes=1  RuntimeRangeChecks=off
  Selector20 : Selector  NumberOfDimensions=2  InputPortWidth=3  IndexOptions=Index vector (dialog),Index vector (dialog)  Indices=[2:16],[1:16]  OutputSizes=1,1  RuntimeRangeChecks=off
  Selector21 : Selector  NumberOfDimensions=2  InputPortWidth=3  IndexOptions=Index vector (dialog),Index vector (dialog)  Indices=[1 2 3 9 10 11],[1:16]  OutputSizes=1,1  RuntimeRangeChecks=off
  Selector22 : Selector  NumberOfDimensions=2  InputPortWidth=16*16  IndexOptions=Index vector (dialog),Index vector (dialog)  Indices=1,[1:16]  OutputSizes=1,1  RuntimeRangeChecks=off
  Selector23 : Selector  NumberOfDimensions=2  InputPortWidth=16*16  IndexOptions=Index vector (dialog),Index vector (dialog)  Indices=2,[1:16]  OutputSizes=1,1  RuntimeRangeChecks=off
  Selector24 : Selector  NumberOfDimensions=2  InputPortWidth=16*16  IndexOptions=Index vector (dialog),Index vector (dialog)  Indices=3,[1:16]  OutputSizes=1,1  RuntimeRangeChecks=off
  Selector25 : Selector  NumberOfDimensions=2  InputPortWidth=16*16  IndexOptions=Index vector (dialog),Index vector (dialog)  Indices=4,[1:16]  OutputSizes=1,1  RuntimeRangeChecks=off
  Selector26 : Selector  NumberOfDimensions=2  InputPortWidth=16*16  IndexOptions=Index vector (dialog),Index vector (dialog)  Indices=5,[1:16]  OutputSizes=1,1  RuntimeRangeChecks=off
  Selector27 : Selector  NumberOfDimensions=2  InputPortWidth=16*16  IndexOptions=Index vector (dialog),Index vector (dialog)  Indices=6,[1:16]  OutputSizes=1,1  RuntimeRangeChecks=off
  Selector28 : Selector  NumberOfDimensions=2  InputPortWidth=16*16  IndexOptions=Index vector (dialog),Index vector (dialog)  Indices=7,[1:16]  OutputSizes=1,1  RuntimeRangeChecks=off
  Selector29 : Selector  NumberOfDimensions=2  InputPortWidth=16*16  IndexOptions=Index vector (dialog),Index vector (dialog)  Indices=8,[1:16]  OutputSizes=1,1  RuntimeRangeChecks=off
  Selector3 : Selector  InputPortWidth=16*16  IndexOptions=Index vector (dialog)  Indices=[1:16]+16*3  OutputSizes=1  RuntimeRangeChecks=off
  Selector30 : Selector  NumberOfDimensions=2  InputPortWidth=16*16  IndexOptions=Index vector (dialog),Index vector (dialog)  Indices=9,[1:16]  OutputSizes=1,1  RuntimeRangeChecks=off
  Selector31 : Selector  NumberOfDimensions=2  InputPortWidth=16*16  IndexOptions=Index vector (dialog),Index vector (dialog)  Indices=10,[1:16]  OutputSizes=1,1  RuntimeRangeChecks=off
  Selector32 : Selector  NumberOfDimensions=2  InputPortWidth=16*16  IndexOptions=Index vector (dialog),Index vector (dialog)  Indices=11,[1:16]  OutputSizes=1,1  RuntimeRangeChecks=off
  Selector33 : Selector  NumberOfDimensions=2  InputPortWidth=16*16  IndexOptions=Index vector (dialog),Index vector (dialog)  Indices=12,[1:16]  OutputSizes=1,1  RuntimeRangeChecks=off
  Selector34 : Selector  NumberOfDimensions=2  InputPortWidth=16*16  IndexOptions=Index vector (dialog),Index vector (dialog)  Indices=13,[1:16]  OutputSizes=1,1  RuntimeRangeChecks=off
  Selector35 : Selector  NumberOfDimensions=2  InputPortWidth=16*16  IndexOptions=Index vector (dialog),Index vector (dialog)  Indices=14,[1:16]  OutputSizes=1,1  RuntimeRangeChecks=off
  Selector36 : Selector  NumberOfDimensions=2  InputPortWidth=16*16  IndexOptions=Index vector (dialog),Index vector (dialog)  Indices=15,[1:16]  OutputSizes=1,1  RuntimeRangeChecks=off
  Selector37 : Selector  NumberOfDimensions=2  InputPortWidth=16*16  IndexOptions=Index vector (dialog),Index vector (dialog)  Indices=16,[1:16]  OutputSizes=1,1  RuntimeRangeChecks=off
  Selector38 : Selector  InputPortWidth=16*16  IndexOptions=Index vector (dialog)  Indices=[1:16]  OutputSizes=1  RuntimeRangeChecks=off
  Selector4 : Selector  InputPortWidth=16*16  IndexOptions=Index vector (dialog)  Indices=[1:16]+16*4  OutputSizes=1  RuntimeRangeChecks=off
  Selector5 : Selector  InputPortWidth=16*16  IndexOptions=Index vector (dialog)  Indices=[1:16]+16*5  OutputSizes=1  RuntimeRangeChecks=off
  Selector6 : Selector  InputPortWidth=16*16  IndexOptions=Index vector (dialog)  Indices=[1:16]+16*6  OutputSizes=1  RuntimeRangeChecks=off
  Selector7 : Selector  InputPortWidth=16*16  IndexOptions=Index vector (dialog)  Indices=[1:16]+16*7  OutputSizes=1  RuntimeRangeChecks=off
  Selector8 : Selector  InputPortWidth=16*16  IndexOptions=Index vector (dialog)  Indices=[1:16]+16*8  OutputSizes=1  RuntimeRangeChecks=off
  Selector9 : Selector  InputPortWidth=16*16  IndexOptions=Index vector (dialog)  Indices=[1:16]+16*9  OutputSizes=1  RuntimeRangeChecks=off
  Signal Specification : SignalSpecification  Dimensions=[16,1]
  Signal Specification1 : SignalSpecification  Dimensions=[1,16]
  add1 : Subsystem
  add2 : Subsystem
  add3 : Subsystem
  add4 : Subsystem
  dot1 : Subsystem  TreatAsAtomicUnit=on
  dot2 : Subsystem  TreatAsAtomicUnit=on
  dot3 : Subsystem  TreatAsAtomicUnit=on
  dot4 : Subsystem  TreatAsAtomicUnit=on
  mult1 : Subsystem
  mult2 : Subsystem
  mult25_recip : Math  Operator=reciprocal  OutputSignalType=real  OutDataTypeStr=single
  mult3 : Subsystem
  mult4 : Subsystem
  multdiv1 : Subsystem
  y_port : Outport
  Dmod : Outport  Port=2
  wires:
  Aflat/1 -> [Aflat], Selector10/1, Selector11/1, Selector12/1, Selector13/1, Selector15/1, Selector14/1, Selector9/1, Selector8/1, Selector7/1, Selector6/1, Selector5/1, Selector4/1, Selector3/1, Selector2/1, Selector1/1, Selector/1
  Divide1/1 -> Add1/2
  mult25_recip/1 -> Divide4/1, Mux3/1  "temp"
  Selector17/1 -> Signal Specification/1
  Constant1/1 -> Add1/1
  Selector18/1 -> Mux3/2
  Selector20/1 -> Matrix Concatenate/2  "DxRow"
  Mux3/1 -> Demux/1  "DxCol"
  Selector16/1 -> Divide1/2
  Constant2/1 -> Matrix Concatenate/1
  Matrix Concatenate/1 -> Add2/2
  Add1/1 -> mult25_recip/1
  [Yrl] -> Divide4/2
  [Aflat] -> Selector17/1, Selector38/1, Selector16/1
  Selector38/1 -> Signal Specification1/1
  Selector8/1 -> add3/2(In1)
  Selector9/1 -> add3/4(In4)
  Selector10/1 -> add3/6(In7)
  Selector11/1 -> add3/8(In10)
  Selector12/1 -> add4/2(In1)
  Selector13/1 -> add4/4(In4)
  Selector14/1 -> add4/6(In7)
  Selector15/1 -> add4/8(In10)
  Selector30/1 -> add3/3(In2)
  Selector31/1 -> add3/5(In5)
  Selector32/1 -> add3/7(In8)
  Selector33/1 -> add3/9(In11)
  Selector34/1 -> add4/3(In2)
  Selector35/1 -> add4/5(In5)
  Selector36/1 -> add4/7(In8)
  Selector37/1 -> add4/9(In11)
  [YrldxRowCol] -> Selector23/1, Selector26/1, Selector27/1, Selector28/1, Selector29/1, Selector30/1, Selector31/1, Selector32/1, Selector33/1, Selector34/1, Selector35/1, Selector37/1, Selector36/1, Selector25/1, Selector24/1, Selector22/1
  D_SOC/1 -> Selector20/1, Selector19/1
  Ysw/1 -> [Yrl], Divide1/1
  [D_update] -> add1/1(E)
  Add2/1 -> Selector21/1
  Selector21/1 -> Dmod/1  "DxRow"
  Signal Specification1/1 -> mult2/2(In2), mult2/4(In4), mult2/6(In6), mult3/2(In2), mult3/6(In6), mult4/8(In8), mult4/6(In6), mult4/4(In4), mult4/2(In2), mult3/8(In8), mult3/4(In4), mult2/8(In8), mult1/8(In8), mult1/6(In6), mult1/4(In4), mult1/2(In2)
  Matrix Concatenate2/1 -> [YrldxRowCol], Add2/1
  Mux4/1 -> y_port/1
  x_port/1 -> dot1/7(In7), dot2/1(In1), dot3/1(In1), dot4/1(In1), dot3/7(In7), dot3/5(In5), dot3/3(In3), dot2/7(In7), dot2/5(In5), dot2/3(In3), dot1/5(In5), dot1/3(In3), dot1/1(In1)
  dot1/1(Out1) -> Mux4/1
  dot1/2(Out2) -> Mux4/2
  dot1/3(Out3) -> Mux4/3
  dot1/4(Out4) -> Mux4/4
  add2/1(y) -> dot2/2(y)
  add2/2(y1) -> dot2/4(y1)
  add2/3(y2) -> dot2/6(y2)
  add2/4(y3) -> dot2/8(y3)
  dot2/1(Out1) -> Mux4/5
  dot2/2(Out2) -> Mux4/6
  dot2/3(Out3) -> Mux4/7
  dot2/4(Out4) -> Mux4/8
  add3/1(y) -> dot3/2(y)
  add3/2(y1) -> dot3/4(y1)
  add3/3(y2) -> dot3/6(y2)
  add3/4(y3) -> dot3/8(y3)
  dot3/1(Out1) -> Mux4/9
  dot3/2(Out2) -> Mux4/10
  dot3/3(Out3) -> Mux4/11
  dot3/4(Out4) -> Mux4/12
  add4/1(y) -> dot4/2(In2)
  add4/2(y1) -> dot4/3(In3)
  add4/3(y2) -> dot4/4(In4)
  add4/4(y3) -> dot4/5(In5)
  dot4/1(Out1) -> Mux4/13
  dot4/2(Out2) -> Mux4/14
  dot4/3(Out3) -> Mux4/15
  dot4/4(Out4) -> Mux4/16
  trig/1 -> [D_update]
  add1/1(y) -> dot1/2(In2)
  add1/2(y1) -> dot1/4(In4)
  add1/3(y2) -> dot1/6(In6)
  add1/4(y3) -> dot1/8(In8)
  [D_update] -> add2/1(E)
  Selector29/1 -> add2/9(In11)
  Selector28/1 -> add2/7(In8)
  Selector27/1 -> add2/5(In5)
  Selector26/1 -> add2/3(In2)
  Selector4/1 -> add2/2(In1)
  Selector5/1 -> add2/4(In4)
  Selector6/1 -> add2/6(In7)
  Selector7/1 -> add2/8(In10)
  Constant3/1 -> add1/2(In1)
  Selector23/1 -> add1/4(In4)
  Selector24/1 -> add1/6(In7)
  Selector25/1 -> add1/8(In10)
  Selector3/1 -> add1/9(In11)
  Selector2/1 -> add1/7(In8)
  Selector1/1 -> add1/5(In5)
  Selector/1 -> add1/3(In2)
  [D_update] -> add3/1(E)
  [D_update] -> add4/1(E)
  Demux/1 -> mult1/1(In1)
  Demux/2 -> mult1/3(In3)
  Demux/3 -> mult1/5(In5)
  Demux/4 -> mult1/7(In7)
  mult1/1(DxCol*DxRow) -> Matrix Concatenate2/1
  mult1/2(DxCol*DxRow1) -> Matrix Concatenate2/2
  mult1/3(DxCol*DxRow2) -> Matrix Concatenate2/3
  mult1/4(DxCol*DxRow3) -> Matrix Concatenate2/4
  mult2/1(DxCol*DxRow) -> Matrix Concatenate2/5
  mult2/2(DxCol*DxRow1) -> Matrix Concatenate2/6
  mult2/3(DxCol*DxRow2) -> Matrix Concatenate2/7
  mult2/4(DxCol*DxRow3) -> Matrix Concatenate2/8
  Demux/5 -> mult2/1(In1)
  Demux/6 -> mult2/3(In3)
  Demux/7 -> mult2/5(In5)
  Demux/8 -> mult2/7(In7)
  mult3/1(DxCol*DxRow) -> Matrix Concatenate2/9
  mult3/2(DxCol*DxRow1) -> Matrix Concatenate2/10
  mult3/3(DxCol*DxRow2) -> Matrix Concatenate2/11
  mult3/4(DxCol*DxRow3) -> Matrix Concatenate2/12
  Demux/9 -> mult3/1(In1)
  Demux/10 -> mult3/3(In3)
  Demux/11 -> mult3/5(In5)
  Demux/12 -> mult3/7(In7)
  mult4/1(DxCol*DxRow) -> Matrix Concatenate2/13
  mult4/2(DxCol*DxRow1) -> Matrix Concatenate2/14
  mult4/3(DxCol*DxRow2) -> Matrix Concatenate2/15
  mult4/4(DxCol*DxRow3) -> Matrix Concatenate2/16
  Demux/13 -> mult4/1(In1)
  Demux/14 -> mult4/3(In3)
  Demux/15 -> mult4/5(In5)
  Demux/16 -> mult4/7(In7)
  Divide4/1 -> multdiv1/1(In1)
  Signal Specification/1 -> multdiv1/2(In2)
  multdiv1/1(DxCol_) -> Selector18/1

== system InductionHeating_bb_4/soc16/MATE 2-level inverter SWFHIZ (3p) ==
  g_up : Inport
  g_lo : Inport  Port=2
  inverter_pram : Inport  Port=3
  Vdc : Inport  Port=4
  Iac(1) : Inport  Port=5
  SW : Subsystem  Commented=on  AncestorBlock=simetranss/FPGA/MATE 2-level inverter SWFHIZ/SW
  SW1 : Subsystem
  Vac(1) : Outport
  Idc : Outport  Port=2
  wires:
  SW1/1(Idc) -> Idc/1
  SW1/2(Vac) -> Vac(1)/1
  g_up/1 -> SW1/1(gu)
  g_lo/1 -> SW1/2(gl)
  Vdc/1 -> SW1/3(Vdc)
  Iac(1)/1 -> SW1/4(Iac)
  inverter_pram/1 -> SW1/5(params)

== system InductionHeating_bb_4/soc16/PWM_Generator at Ts ==
  note: must change deadtime because integrator reset must be scalar
  PWMsteps : Inport
  PWMstepsON : Inport  Port=2
  deatime(s) : Inport  Port=3
  enable : Inport  Port=4
  Constant : Constant  Value=[0 0]  OutDataTypeStr=boolean  SampleTime=Ts
  Data Type Conversion1 : DataTypeConversion  Commented=on  OutDataTypeStr=single  RndMeth=Nearest  SaturateOnIntegerOverflow=off
  Discrete-Time Integrator : DiscreteIntegrator  Commented=on  gainval=1  ExternalReset=level  SampleTime=Ts  LimitOutput=on  ICPrevOutput=DiscIntNeverNeededParam  ICPrevScaledInput=DiscIntNeverNeededParam
  Logical Operator1 : Logic  Operator=NOT  AllPortsSameDT=off  OutDataTypeStr=boolean
  Logical Operator2 : Logic  Commented=on  AllPortsSameDT=off  OutDataTypeStr=boolean
  Logical Operator3 : Logic  Commented=on  Operator=NOT  AllPortsSameDT=off  OutDataTypeStr=boolean
  Mux1 : Mux  Inputs=2
  PWM generator : Subsystem
  Relational Operator1 : RelationalOperator  Commented=on  Operator=>  OutDataTypeStr=boolean  RndMeth=Simplest  InputSameDT=off
  Switch : Switch  Criteria=u2 ~= 0  SaturateOnIntegerOverflow=off  InputSameDT=off
  gate : Outport  VectorParamsAs1DForOutWhenUnconnected=off
  wires:
  deatime(s)/1 -> Relational Operator1/2
  Data Type Conversion1/1 -> Discrete-Time Integrator/1  "Simulink-PS Converter1"
  Mux1/1 -> Logical Operator3/1, Data Type Conversion1/1, Switch/1, Logical Operator2/2
  Logical Operator1/1 -> Mux1/2
  Logical Operator3/1 -> Discrete-Time Integrator/2
  Relational Operator1/1 -> Logical Operator2/1
  Discrete-Time Integrator/1 -> Relational Operator1/1
  PWM generator/1(pulse) -> Logical Operator1/1, Mux1/1
  PWMsteps/1 -> PWM generator/1(steps)
  PWMstepsON/1 -> PWM generator/2(stepON)
  Switch/1 -> gate/1
  enable/1 -> Switch/2
  Constant/1 -> Switch/3
